simulink model "lab4_pid"  (R2025b)
settings: Solver=ode45  StartTime=0.0  StopTime=25  MaxStep=0.02  RelTol=1e-3
undefined symbols (not defined in the file): noiseVar, num1, num2, num3, T, T1, T2p
settings Model: Creator=Nickolay  LastModifiedBy=Nickolay

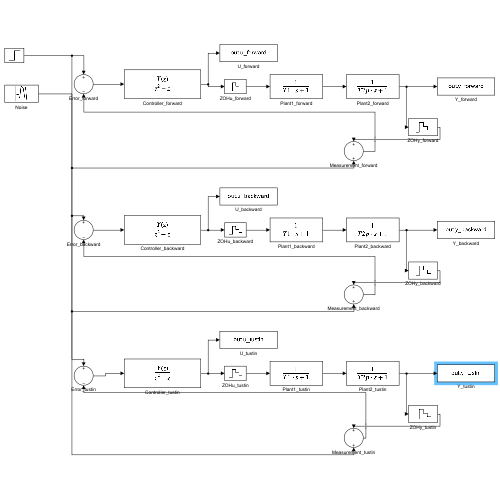
[thumbnail: Simulink's stored preview of the top-level diagram]
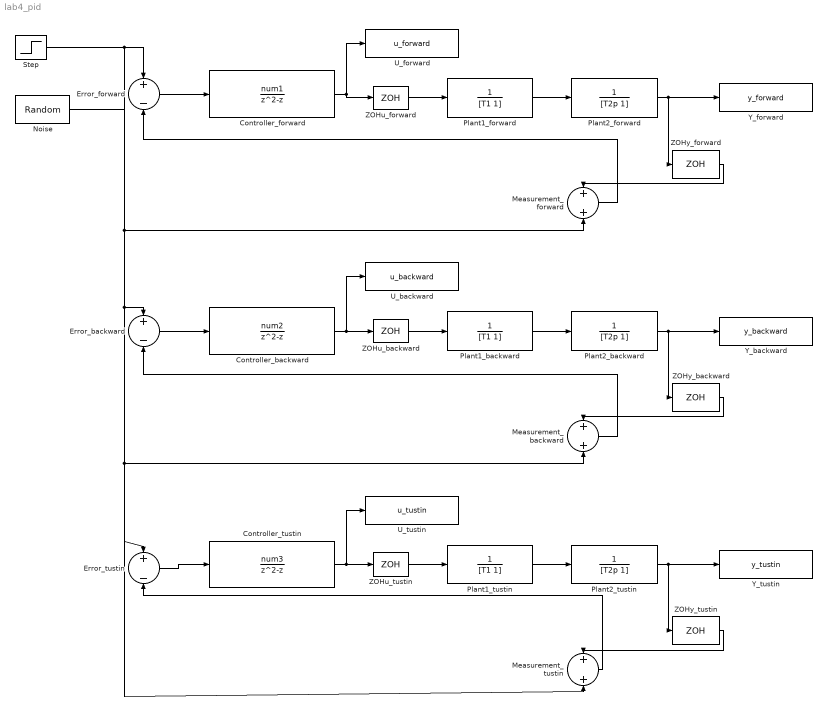
== system lab4_pid ==
  Controller_backward : DiscreteTransferFcn  Numerator=num2  Denominator=[1 -1 0]  SampleTime=T
  Controller_forward : DiscreteTransferFcn  Numerator=num1  Denominator=[1 -1 0]  SampleTime=T
  Controller_tustin : DiscreteTransferFcn  Numerator=num3  Denominator=[1 -1 0]  SampleTime=T
  Error_backward : Sum  Inputs=+-
  Error_forward : Sum  Inputs=+-
  Error_tustin : Sum  Inputs=+-
  Measurement_backward : Sum
  Measurement_forward : Sum
  Measurement_tustin : Sum
  Noise : RandomNumber  Variance=noiseVar  Seed=42  SampleTime=T
  Plant1_backward : TransferFcn  Denominator=[T1 1]
  Plant1_forward : TransferFcn  Denominator=[T1 1]
  Plant1_tustin : TransferFcn  Denominator=[T1 1]
  Plant2_backward : TransferFcn  Denominator=[T2p 1]
  Plant2_forward : TransferFcn  Denominator=[T2p 1]
  Plant2_tustin : TransferFcn  Denominator=[T2p 1]
  Step : Step  Time=0  SampleTime=0
  U_backward : ToWorkspace  VariableName=u_backward  SaveFormat=Timeseries  SampleTime=-1
  U_forward : ToWorkspace  VariableName=u_forward  SaveFormat=Timeseries  SampleTime=-1
  U_tustin : ToWorkspace  VariableName=u_tustin  SaveFormat=Timeseries  SampleTime=-1
  Y_backward : ToWorkspace  VariableName=y_backward  SaveFormat=Timeseries  SampleTime=-1
  Y_forward : ToWorkspace  VariableName=y_forward  SaveFormat=Timeseries  SampleTime=-1
  Y_tustin : ToWorkspace  VariableName=y_tustin  SaveFormat=Timeseries  SampleTime=-1
  ZOHu_backward : ZeroOrderHold  SampleTime=T
  ZOHu_forward : ZeroOrderHold  SampleTime=T
  ZOHu_tustin : ZeroOrderHold  SampleTime=T
  ZOHy_backward : ZeroOrderHold  SampleTime=T
  ZOHy_forward : ZeroOrderHold  SampleTime=T
  ZOHy_tustin : ZeroOrderHold  SampleTime=T
  wires:
  Step/1 -> Error_backward/1, Error_tustin/1, Error_forward/1
  Error_forward/1 -> Controller_forward/1
  Controller_forward/1 -> ZOHu_forward/1, U_forward/1
  ZOHu_forward/1 -> Plant1_forward/1
  Plant1_forward/1 -> Plant2_forward/1
  Plant2_forward/1 -> Y_forward/1, ZOHy_forward/1
  ZOHy_forward/1 -> Measurement_forward/1
  Noise/1 -> Measurement_backward/2, Measurement_tustin/2, Measurement_forward/2
  Measurement_forward/1 -> Error_forward/2
  Error_backward/1 -> Controller_backward/1
  Controller_backward/1 -> ZOHu_backward/1, U_backward/1
  ZOHu_backward/1 -> Plant1_backward/1
  Plant1_backward/1 -> Plant2_backward/1
  Plant2_backward/1 -> Y_backward/1, ZOHy_backward/1
  ZOHy_backward/1 -> Measurement_backward/1
  Measurement_backward/1 -> Error_backward/2
  Error_tustin/1 -> Controller_tustin/1
  Controller_tustin/1 -> ZOHu_tustin/1, U_tustin/1
  ZOHu_tustin/1 -> Plant1_tustin/1
  Plant1_tustin/1 -> Plant2_tustin/1
  Plant2_tustin/1 -> Y_tustin/1, ZOHy_tustin/1
  ZOHy_tustin/1 -> Measurement_tustin/1
  Measurement_tustin/1 -> Error_tustin/2
